simulink model "MotorGenerator2_Component_harness_model"  (R2023a)
settings: Solver=daessc  StartTime=0.0  StopTime=200  RelTol=1e-3  AbsTol=1e-3
PreLoadFcn:
  | MotorGenerator2_Component_harness_setup
undefined symbols (not defined in the file or in its folder): batteryHighVoltage, initial, Minus, motorGenerator2, Plus
libraries: fl_lib x18, nesl_utility x14, sdl_lib x1
settings Model: Creator=isaacito  LastModifiedBy=isaacito
settings SolverCC: AutoScaleAbsTol=off  AlgebraicLoopSolver=TrustRegion
settings DataIOCC: DSMLogging=off
settings OptimizationCC: ReuseModelBlockBuffer=off
settings DebuggingCC: UnconnectedInputMsg=warning  UnconnectedOutputMsg=warning  UnconnectedLineMsg=warning  SymbolicDimsDataTypeCodeGenerationDiagnostic=none
settings ModelReferenceCC: EnableRefExpFcnMdlSchedulingChecks=on
settings SFSimCC: CustomCodeUndefinedFunction=UseInterfaceOnly
settings RTWCC: DLArmComputeVersion=19.05
settings SimscapeCC: SimscapeLogType=all  SimscapeLogSimulationStatistics=on  SimscapeLogLimitData=off  SimscapeLogDataHistory=10000

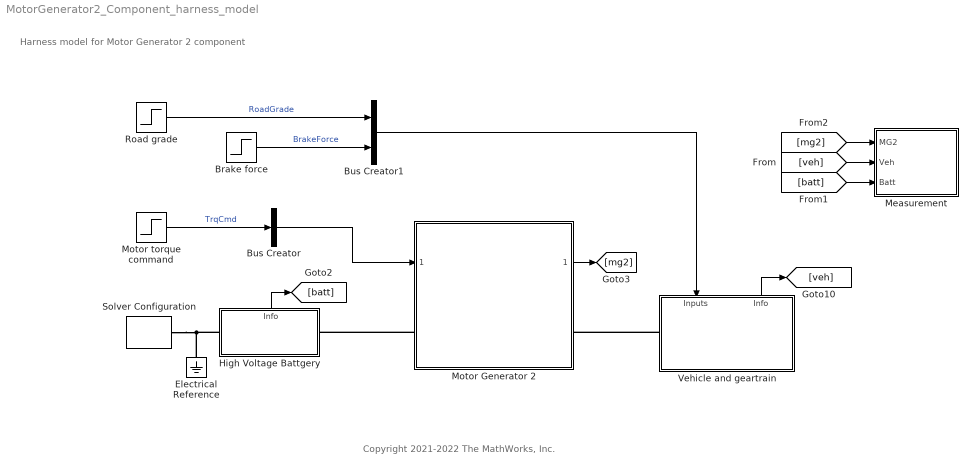
== system MotorGenerator2_Component_harness_model ==
  note: Copyright 2021-2022 The MathWorks, Inc.
  note: Harness model for Motor Generator 2 component
  Brake force : Step  After=0  SampleTime=0
      settings: AttributesFormatString=|
      | Before: %<Before>
      | Time: %<Time>
      | After: %<After>
  Bus Creator : BusCreator  Inputs=1
  Bus Creator1 : BusCreator  Inputs=2
  Electrical Reference : fl_lib/Electrical/Electrical Elements/Electrical Reference
  High Voltage Battgery : Subsystem
      settings: PortSchema="{\"entries\":[{\"content\":{\"sides\":[{\"content\":{\"connectorIds\":[\"LConn1\"]},\"type\":\"ConnectorPlacement.EquallySpacedRectSide\",\"uuid\":\"8acd7e9a-bb08-4de6-aa14-0989ebba81b9\"},{\"content\":{\"connectorIds\":[\"RConn1\"],\"side\":\"RIGHT\"},\"type\":\"ConnectorPlacement.EquallySpacedRectSide\",\"uuid\":\"f80e1afc-966f-4d6b-84f9-f0b60dd6f20c\"},{\"content\":{\"connectorIds\":[\"Out1\"],\"side\":\"TOP\"},\"type\":\"ConnectorPlacement.EquallySpacedRectSide\",\"uuid\":\"52ccb2b1-bd5e-4dcb-b9b6-0ef03b912c33\"}]},\"type\":\"ConnectorPlacement.EquallySpacedConnector\",\"uuid\":\"b55f48a4-f283-4a77-8513-99b31abb285a\"}],\"packageUris\":[\"http://schema.mathworks.com/mf0/Connector/R2020b\"],\"version\":\"1.0\"}"
  Measurement : Subsystem
  Motor Generator 2 : Subsystem  ReferencedSubsystem=MotorDriveUnit_refsub_Basic  torque_max=motorGenerator2.trqMax_Nm  Value=motorGenerator2.powerMax_kW  Tc=motorGenerator2.responseTime_s  eff=motorGenerator2.efficiency_pct  w_eff=motorGenerator2.spd_eff_rpm  T_eff=motorGenerator2.trq_eff_Nm  thermal_mass=motorGenerator2.thermalMass_J_perK  temperature=initial.MG2_Temperature_K  k=motorGenerator2.dampSpringStiffness_Nm_per_rad  mu_visc=motorGenerator2.dampSpringFriction_Nm_per_rpm  w_tol=smoothing.MG2_dampSpringVelTol_rpm  T=initial.MG2_AirTemp_K
      settings: PortSchema="{\"entries\":[{\"content\":{\"sides\":[{\"content\":{\"connectorIds\":[\"In1\",\"LConn1\"]},\"type\":\"ConnectorPlacement.EquallySpacedRectSide\",\"uuid\":\"02d16a10-ccfb-4288-a5a1-1144159c5ca2\"},{\"content\":{\"connectorIds\":[\"Out1\",\"LConn2\"],\"side\":\"RIGHT\"},\"type\":\"ConnectorPlacement.EquallySpacedRectSide\",\"uuid\":\"b2601986-efe5-4f5e-bd54-3f5cb03e9252\"},{\"content\":{\"connectorIds\":[],\"side\":\"TOP\"},\"type\":\"ConnectorPlacement.EquallySpacedRectSide\",\"uuid\":\"248805f0-4416-4f49-8b0b-c2d3fe77e89e\"}]},\"type\":\"ConnectorPlacement.EquallySpacedConnector\",\"uuid\":\"35449164-35fe-478e-9b2e-66e853caa6da\"}],\"packageUris\":[\"http://schema.mathworks.com/mf0/Connector/R2020b\"],\"version\":\"1.0\"}"
  Motor torque command : Step  Time=50  Before=50  After=100  SampleTime=0
      settings: AttributesFormatString=|
      | Before: %<Before>
      | Time: %<Time>
      | After: %<After>
  Road grade : Step  Time=100  After=7  SampleTime=0
      settings: AttributesFormatString=|
      | Before: %<Before>
      | Time: %<Time>
      | After: %<After>
  Solver Configuration : nesl_utility/Solver Configuration  PhysicalDomain=network_engine_domain  SubClassName=solver  LeftPortType=input  RightPortType=generic  Tones=[]  Harmonics=[]  SimulateNoise=off  Profile=off  UseLocalSampling=off  EnableSwitchedLinearOptims=on  FrequencyDomain=off  UseCCode=off  RelTol=0.001  AbsTol=1e-06  MinStep=1e-09  ToWorkspace=off  RevertToSquareIcSolve=off  NumHomotopyIterations=100  PhasorMode=off  PhasorModeNumHarmonics=1  ConsistencySolver=NEWTON_FTOL  IndexReductionMethod=DerivativeReplacement  DoDC=off  ResidualTolerance=1e-09  ConsistencyTolSource=GLOBAL  ConsistencyAbsTol=0.001  ConsistencyRelTol=0.001  ConsistencyTolFactor=0.001  UseLocalSolver=off  LocalSolverChoice=NE_BACKWARD_EULER_ADVANCER  ResolveIndetEquations=on  FunctionEvalNumThread=1  LocalSolverSampleTime=0.001  DoFixedCost=off  MaxNonlinIter=3  MaxModeIter=2  ComputeImpulses=off  ImpulseIterations=2  LinearAlgebra=auto  LinearAlgebraNumThread=0  EquationFormulation=NE_TIME_EF  DelaysMemoryBudget=1024  AutomaticFiltering=on  FilteringTimeConstant=0.001  PartitionStorageMethod=AS_NEEDED  PartitionMemoryBudget=1024  PartitionMethod=ROBUST
      settings: AttributesFormatString=Local solver %<UseLocalSolver>
  Vehicle and geartrain : Subsystem
      settings: PortSchema="{\"entries\":[{\"content\":{\"sides\":[{\"content\":{\"connectorIds\":[\"LConn1\"]},\"type\":\"ConnectorPlacement.EquallySpacedRectSide\",\"uuid\":\"26173f4b-7c8a-4f16-9397-bd2703a262c3\"},{\"content\":{\"connectorIds\":[],\"side\":\"RIGHT\"},\"type\":\"ConnectorPlacement.EquallySpacedRectSide\",\"uuid\":\"c1cca5f5-e160-4db7-9272-a3c788f9ef94\"},{\"content\":{\"connectorIds\":[\"In1\",\"Out1\"],\"side\":\"TOP\"},\"type\":\"ConnectorPlacement.EquallySpacedRectSide\",\"uuid\":\"12b52f59-061a-44b9-b00e-a084783c45fb\"}]},\"type\":\"ConnectorPlacement.EquallySpacedConnector\",\"uuid\":\"a6613901-d795-4b91-ba16-2f1b373021b5\"}],\"packageUris\":[\"http://schema.mathworks.com/mf0/Connector/R2020b\"],\"version\":\"1.0\"}"
  wires:
  High Voltage Battgery/1(Info) -> [batt]
  Motor Generator 2/1 -> [mg2]
  Vehicle and geartrain/1(Info) -> [veh]
  [veh] -> Measurement/2(Veh)
  [mg2] -> Measurement/1(MG2)
  [batt] -> Measurement/3(Batt)
  Motor torque command/1 -> Bus Creator/1  "TrqCmd"
  Bus Creator/1 -> Motor Generator 2/1
  Road grade/1 -> Bus Creator1/1  "RoadGrade"
  Brake force/1 -> Bus Creator1/2  "BrakeForce"
  Bus Creator1/1 -> Vehicle and geartrain/1(Inputs)
  connections:
  High Voltage Battgery/LConn1 -- Solver Configuration/RConn1 -- Electrical Reference/LConn1
  Motor Generator 2/LConn1 -- High Voltage Battgery/RConn1
  Vehicle and geartrain/LConn1 -- Motor Generator 2/LConn2

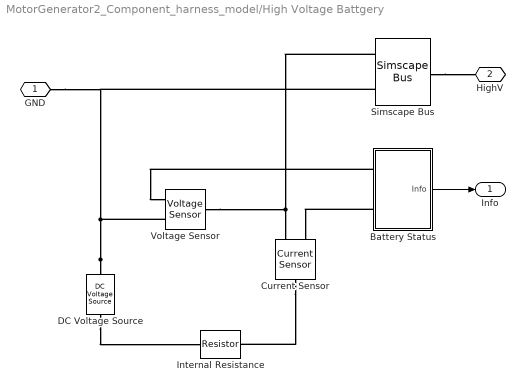
== system MotorGenerator2_Component_harness_model/High Voltage Battgery ==
  Battery Status : Subsystem
  Current Sensor : fl_lib/Electrical/Electrical Sensors/Current Sensor
  DC Voltage Source : fl_lib/Electrical/Electrical Sources/DC Voltage Source  v0=batteryHighVoltage.voltage_V V
      settings: AttributesFormatString=%<v0> [%<v0_unit>]
  Internal Resistance : fl_lib/Electrical/Electrical Elements/Resistor  R=batteryHighVoltage.internal_R_Ohm Ohm  i_specify=off  i_priority=High  i=0 A  i_nominal_specify=off  i_nominal_unit=A  i_nominal_value=1  v_specify=off  v_priority=High  v=0 V  v_nominal_specify=off  v_nominal_unit=V  v_nominal_value=1
      settings: AttributesFormatString=%<R> [%<R_unit>]
  Simscape Bus : SimscapeBus  HierarchyStrings=Plus;Minus  ConnectionType=Bus: Bus_HighVoltage
      settings: AttributesFormatString=%<ConnectionType>
  Voltage Sensor : fl_lib/Electrical/Electrical Sensors/Voltage Sensor
  GND : PMIOPort  Side=Left
  HighV : PMIOPort  Port=2  Side=Right
  Info : Outport
  wires:
  Battery Status/1(Info) -> Info/1
  connections:
  DC Voltage Source/RConn1 -- Simscape Bus/LConn2 -- GND/RConn1 -- Voltage Sensor/RConn2
  Simscape Bus/LConn1 -- Voltage Sensor/LConn1 -- Current Sensor/RConn2
  Battery Status/LConn2 -- Current Sensor/RConn1
  Simscape Bus/RConn1 -- HighV/RConn1
  Current Sensor/LConn1 -- Internal Resistance/RConn1
  DC Voltage Source/LConn1 -- Internal Resistance/LConn1
  Battery Status/LConn1 -- Voltage Sensor/RConn1

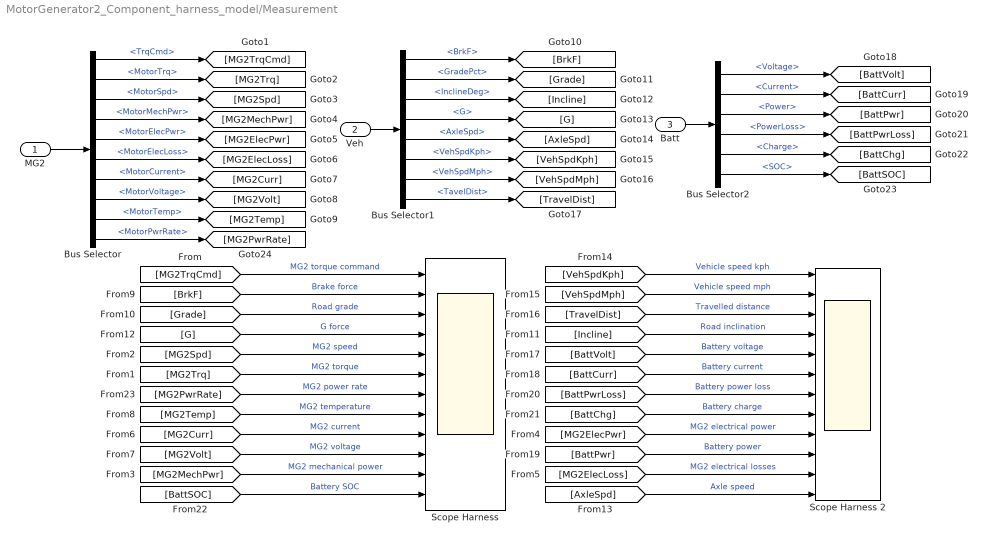
== system MotorGenerator2_Component_harness_model/Measurement ==
  MG2 : Inport
  Veh : Inport  Port=2
  Batt : Inport  Port=3
  Bus Selector : BusSelector  OutputSignals=TrqCmd,MotorTrq,MotorSpd,MotorMechPwr,MotorElecPwr,MotorElecLoss,MotorCurrent,MotorVoltage,MotorTemp,MotorPwrRate
  Bus Selector1 : BusSelector  OutputSignals=BrkF,GradePct,InclineDeg,G,AxleSpd,VehSpdKph,VehSpdMph,TavelDist
  Bus Selector2 : BusSelector  OutputSignals=Voltage,Current,Power,PowerLoss,Charge,SOC
  Scope Harness : Scope  NumInputPorts=12
  Scope Harness 2 : Scope  NumInputPorts=12
  wires:
  Veh/1 -> Bus Selector1/1
  MG2/1 -> Bus Selector/1
  Bus Selector/1 -> [MG2TrqCmd]  "<TrqCmd>"
  Bus Selector/2 -> [MG2Trq]  "<MotorTrq>"
  Bus Selector/3 -> [MG2Spd]  "<MotorSpd>"
  Bus Selector/4 -> [MG2MechPwr]  "<MotorMechPwr>"
  Bus Selector/5 -> [MG2ElecPwr]  "<MotorElecPwr>"
  Bus Selector/6 -> [MG2ElecLoss]  "<MotorElecLoss>"
  Bus Selector/7 -> [MG2Curr]  "<MotorCurrent>"
  Bus Selector/8 -> [MG2Volt]  "<MotorVoltage>"
  Bus Selector/9 -> [MG2Temp]  "<MotorTemp>"
  Batt/1 -> Bus Selector2/1
  Bus Selector1/1 -> [BrkF]  "<BrkF>"
  Bus Selector1/2 -> [Grade]  "<GradePct>"
  Bus Selector1/3 -> [Incline]  "<InclineDeg>"
  Bus Selector1/4 -> [G]  "<G>"
  Bus Selector1/5 -> [AxleSpd]  "<AxleSpd>"
  Bus Selector1/6 -> [VehSpdKph]  "<VehSpdKph>"
  Bus Selector1/7 -> [VehSpdMph]  "<VehSpdMph>"
  Bus Selector1/8 -> [TravelDist]  "<TavelDist>"
  Bus Selector2/1 -> [BattVolt]  "<Voltage>"
  Bus Selector2/2 -> [BattCurr]  "<Current>"
  Bus Selector2/3 -> [BattPwr]  "<Power>"
  Bus Selector2/4 -> [BattPwrLoss]  "<PowerLoss>"
  Bus Selector2/5 -> [BattChg]  "<Charge>"
  Bus Selector2/6 -> [BattSOC]  "<SOC>"
  [MG2TrqCmd] -> Scope Harness/1  "MG2 torque command"
  [BrkF] -> Scope Harness/2  "Brake force"
  [Grade] -> Scope Harness/3  "Road grade"
  [G] -> Scope Harness/4  "G force"
  [MG2Spd] -> Scope Harness/5  "MG2 speed"
  [MG2Trq] -> Scope Harness/6  "MG2 torque"
  [MG2Temp] -> Scope Harness/8  "MG2 temperature"
  [MG2Curr] -> Scope Harness/9  "MG2 current"
  [MG2Volt] -> Scope Harness/10  "MG2 voltage"
  [BattSOC] -> Scope Harness/12  "Battery SOC"
  [VehSpdKph] -> Scope Harness 2/1  "Vehicle speed kph"
  [VehSpdMph] -> Scope Harness 2/2  "Vehicle speed mph"
  [TravelDist] -> Scope Harness 2/3  "Travelled distance"
  [Incline] -> Scope Harness 2/4  "Road inclination"
  [BattVolt] -> Scope Harness 2/5  "Battery voltage"
  [BattCurr] -> Scope Harness 2/6  "Battery current"
  [BattPwrLoss] -> Scope Harness 2/7  "Battery power loss"
  [BattChg] -> Scope Harness 2/8  "Battery charge"
  [MG2ElecPwr] -> Scope Harness 2/9  "MG2 electrical power"
  Bus Selector/10 -> [MG2PwrRate]  "<MotorPwrRate>"
  [MG2PwrRate] -> Scope Harness/7  "MG2 power rate"
  [MG2MechPwr] -> Scope Harness/11  "MG2 mechanical power"
  [BattPwr] -> Scope Harness 2/10  "Battery power"
  [MG2ElecLoss] -> Scope Harness 2/11  "MG2 electrical losses"
  [AxleSpd] -> Scope Harness 2/12  "Axle speed"

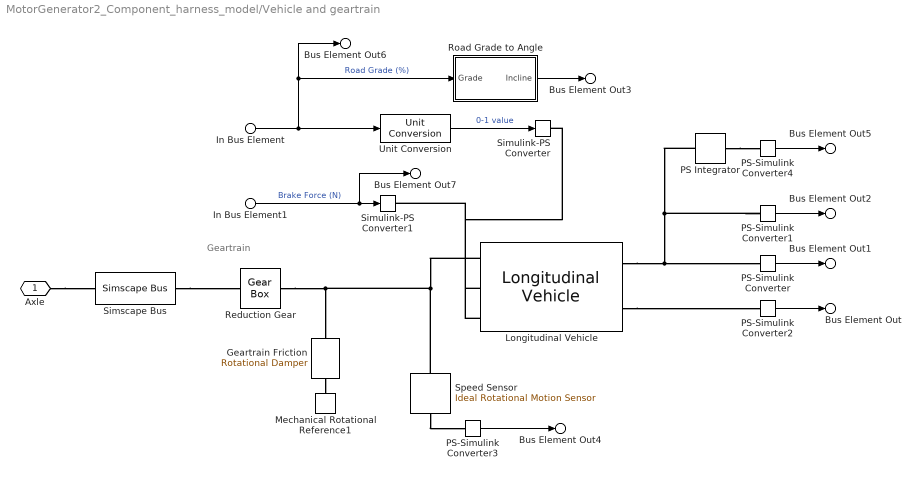
== system MotorGenerator2_Component_harness_model/Vehicle and geartrain ==
  note: Geartrain
  In Bus Element : Inport  PortName=Inputs  Element=RoadGrade
      settings: AttributesFormatString=%<Unit>
  In Bus Element1 : Inport  PortName=Inputs  Element=BrakeForce
      settings: AttributesFormatString=%<Unit>
  Geartrain Friction : fl_lib/Mechanical/Rotational Elements/Rotational Damper  D=0.01 m*N/rpm  w_specify=off  w_priority=None  w=0 rad/s  w_nominal_specify=off  w_nominal_unit=rad/s  w_nominal_value=1  t_specify=off  t_priority=None  t=0 N*m  t_nominal_specify=off  t_nominal_unit=N*m  t_nominal_value=1
      settings: AttributesFormatString=%<D> %<D_unit>
  Longitudinal Vehicle : sdl_lib/Tires & Vehicles/Longitudinal Vehicle  vehParamType=sdl.enum.VehicleParameterizationType.RoadLoad  M_vehicle=1200 kg  R_tireroll=0.3 m  C_tireroll=0.0136  C_airdrag=0.31  A_front=2.3 m^2  A_rl=120 N  B_rl=1.8 N/(m/s)  C_rl=0.389 N/(m/s)^2  g=9.81 m/s^2  V_1=0.3 m/s  w_1=0.01 rad/s  ShowBrakeIn=simscape.enum.onoff.on  ShowSlopeIn=simscape.enum.onoff.on  SlopeInputType=sdl.enum.VehicleLongitudinalRoadSlopeInputType.Grade  ShowWindIn=simscape.enum.onoff.off  ShowGOut=simscape.enum.onoff.on  air_density=1.184 kg/m^3  V_x_specify=on  V_x_priority=High  V_x=initial.vehicle_speed_kph km/hr  V_x_nominal_specify=off  V_x_nominal_unit=m/s  V_x_nominal_value=1  trq_specify=off  trq_priority=None  trq=0 N*m  trq_nominal_specify=off  trq_nominal_unit=N*m  trq_nominal_value=1  w_specify=off  w_priority=None  w=0 rad/s  w_nominal_specify=off  w_nominal_unit=rad/s  w_nominal_value=1
      settings: InternalSimscapePortConfiguration="{\"Bottom\":[],\"Left\":[{\"id\":\"Axle\",\"label\":\"Axle\",\"type\":\"foundation.mechanical.rotational.rotational\"}],\"Right\":[{\"id\":\"v_out\",\"label\":\"VehSpd\",\"type\":\"output\"},{\"id\":\"G_out\",\"label\":\"G\",\"type\":\"output\"}],\"Top\":[{\"id\":\"brkF\",\"label\":\"Brake\",\"type\":\"input\"},{\"id\":\"grade_norm\",\"label\":\"NG\",\"type\":\"input\"}]}"
      settings: AttributesFormatString=|
      | %<V_x> [%<V_x_unit>]
      | Priority: %<V_x_priority>
  Mechanical Rotational Reference1 : fl_lib/Mechanical/Rotational Elements/Mechanical Rotational Reference
  PS Integrator : fl_lib/Physical Signals/Linear Operators/PS Integrator  reset_method=foundation.enum.IntegratorResetSpec.None  initial_condition_spec=foundation.enum.IntegratorICSpec.Internal  saturation_spec=foundation.enum.IntegratorSaturationSpec.None  saturation_source_spec=foundation.enum.IntegratorSaturationSourceSpec.Internal  x0=0 km  xu=inf s  xl=-inf s
      settings: AttributesFormatString=Initial: %<x0> %<x0_unit>
  PS-Simulink Converter : nesl_utility/PS-Simulink Converter  PhysicalDomain=network_engine_domain  SubClassName=ps_output  LeftPortType=input  RightPortType=output  PseudoPeriodic=off  Frequencies=[]  VectorFormat=1-D array  Unit=km/hr  AffineConversion=off
  PS-Simulink Converter1 : nesl_utility/PS-Simulink Converter  PhysicalDomain=network_engine_domain  SubClassName=ps_output  LeftPortType=input  RightPortType=output  PseudoPeriodic=off  Frequencies=[]  VectorFormat=1-D array  Unit=mph  AffineConversion=off
  PS-Simulink Converter2 : nesl_utility/PS-Simulink Converter  PhysicalDomain=network_engine_domain  SubClassName=ps_output  LeftPortType=input  RightPortType=output  PseudoPeriodic=off  Frequencies=[]  VectorFormat=1-D array  Unit=1  AffineConversion=off
  PS-Simulink Converter3 : nesl_utility/PS-Simulink Converter  PhysicalDomain=network_engine_domain  SubClassName=ps_output  LeftPortType=input  RightPortType=output  PseudoPeriodic=off  Frequencies=[]  VectorFormat=1-D array  Unit=rpm  AffineConversion=off
  PS-Simulink Converter4 : nesl_utility/PS-Simulink Converter  PhysicalDomain=network_engine_domain  SubClassName=ps_output  LeftPortType=input  RightPortType=output  PseudoPeriodic=off  Frequencies=[]  VectorFormat=1-D array  Unit=km  AffineConversion=off
  Reduction Gear : fl_lib/Mechanical/Mechanisms/Gear Box  ratio=9  t_in_specify=off  t_in_priority=None  t_in=0 N*m  t_in_nominal_specify=off  t_in_nominal_unit=N*m  t_in_nominal_value=1  t_out_specify=off  t_out_priority=None  t_out=0 N*m  t_out_nominal_specify=off  t_out_nominal_unit=N*m  t_out_nominal_value=1
      settings: AttributesFormatString=%<ratio>
  Road Grade to Angle : Subsystem
  Simscape Bus : SimscapeBus  HierarchyStrings=AngSpd  ConnectionType=Bus: Bus_Rotational
      settings: AttributesFormatString=%<ConnectionType>
  Simulink-PS Converter : nesl_utility/Simulink-PS Converter  PhysicalDomain=network_engine_domain  SubClassName=ps_input  LeftPortType=input  RightPortType=output  PseudoPeriodic=off  Frequencies=[]  NoiseDistribution=none  NoiseParameters=[]  Unit=1  AffineConversion=off  FilteringAndDerivatives=filter  SimscapeFilterOrder=1  InputFilterTimeConstant=0.001  UdotUserProvided=0
  Simulink-PS Converter1 : nesl_utility/Simulink-PS Converter  PhysicalDomain=network_engine_domain  SubClassName=ps_input  LeftPortType=input  RightPortType=output  PseudoPeriodic=off  Frequencies=[]  NoiseDistribution=none  NoiseParameters=[]  Unit=N  AffineConversion=off  FilteringAndDerivatives=filter  SimscapeFilterOrder=1  InputFilterTimeConstant=0.001  UdotUserProvided=0
  Speed Sensor : fl_lib/Mechanical/Mechanical Sensors/Ideal Rotational Motion Sensor  reference=foundation.enum.MeasurementReference.absolute  acceleration_port=false  velocity_port=true  position_port=false  wrap_angle=simscape.enum.onoff.off  offset=0 rad
      settings: InternalSimscapePortConfiguration="{\"Bottom\":[],\"Left\":[{\"id\":\"R\",\"label\":\"R\",\"type\":\"foundation.mechanical.rotational.rotational\"}],\"Right\":[{\"id\":\"W\",\"label\":\"W\",\"type\":\"output\"}],\"Top\":[]}"
  Unit Conversion : UnitConversion  OutputType=Inherit: Inherit via back propagation
  Axle : PMIOPort  Side=Left
  Bus Element Out : Outport  PortName=Info  Element=G
      settings: AttributesFormatString=%<Unit>
  Bus Element Out1 : Outport  PortName=Info  Element=VehSpdKph
      settings: AttributesFormatString=%<Unit>
  Bus Element Out2 : Outport  PortName=Info  Element=VehSpdMph
      settings: AttributesFormatString=%<Unit>
  Bus Element Out3 : Outport  PortName=Info  Element=InclineDeg
      settings: AttributesFormatString=%<Unit>
  Bus Element Out4 : Outport  PortName=Info  Element=AxleSpd
      settings: AttributesFormatString=%<Unit>
  Bus Element Out5 : Outport  PortName=Info  Element=TavelDist
      settings: AttributesFormatString=%<Unit>
  Bus Element Out6 : Outport  PortName=Info  Element=GradePct
      settings: AttributesFormatString=%<Unit>
  Bus Element Out7 : Outport  PortName=Info  Element=BrkF
      settings: AttributesFormatString=%<Unit>
  wires:
  PS-Simulink Converter1/1 -> Bus Element Out2/1
  Unit Conversion/1 -> Simulink-PS Converter/1  "0-1 value"
  In Bus Element1/1 -> Bus Element Out7/1, Simulink-PS Converter1/1  "Brake Force (N)"
  PS-Simulink Converter3/1 -> Bus Element Out4/1
  PS-Simulink Converter/1 -> Bus Element Out1/1
  In Bus Element/1 -> Bus Element Out6/1, Road Grade to Angle/1(Grade), Unit Conversion/1  "Road Grade (%)"
  PS-Simulink Converter2/1 -> Bus Element Out/1
  Road Grade to Angle/1(Incline) -> Bus Element Out3/1
  PS-Simulink Converter4/1 -> Bus Element Out5/1
  connections:
  Longitudinal Vehicle/RConn1 -- PS Integrator/LConn1 -- PS-Simulink Converter1/LConn1 -- PS-Simulink Converter/LConn1
  Longitudinal Vehicle/LConn2 -- Simulink-PS Converter1/RConn1
  Longitudinal Vehicle/LConn3 -- Simulink-PS Converter/RConn1
  Speed Sensor/RConn1 -- PS-Simulink Converter3/LConn1
  Longitudinal Vehicle/RConn2 -- PS-Simulink Converter2/LConn1
  Reduction Gear/RConn1 -- Speed Sensor/LConn1 -- Longitudinal Vehicle/LConn1 -- Geartrain Friction/LConn1
  Simscape Bus/LConn1 -- Reduction Gear/LConn1
  Geartrain Friction/RConn1 -- Mechanical Rotational Reference1/LConn1
  Axle/RConn1 -- Simscape Bus/RConn1
  PS Integrator/RConn1 -- PS-Simulink Converter4/LConn1

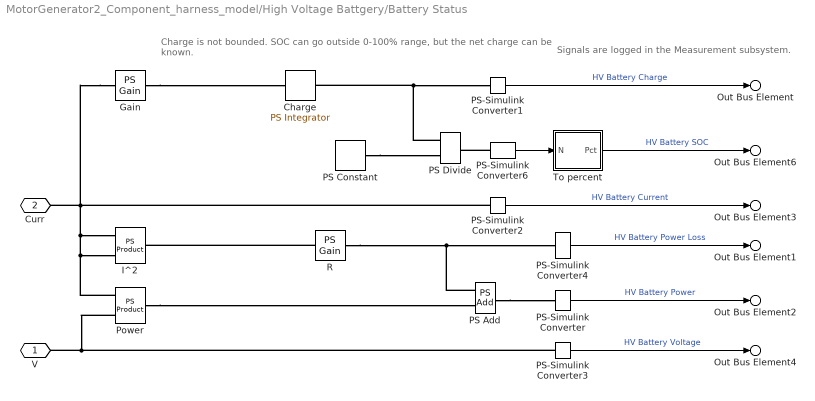
== system MotorGenerator2_Component_harness_model/High Voltage Battgery/Battery Status ==
  note: Signals are logged in the Measurement subsystem.
  note: Charge is not bounded. SOC can go outside 0-100% range,
      | but the net charge can be known.
  Charge : fl_lib/Physical Signals/Linear Operators/PS Integrator  reset_method=foundation.enum.IntegratorResetSpec.None  initial_condition_spec=foundation.enum.IntegratorICSpec.Internal  saturation_spec=foundation.enum.IntegratorSaturationSpec.None  saturation_source_spec=foundation.enum.IntegratorSaturationSourceSpec.Internal  x0=initial.hvBattery_Charge_Ahr A*hr  xu=inf s  xl=-inf s
      settings: AttributesFormatString=%<x0> [%<x0_unit>]
  Gain : fl_lib/Physical Signals/Functions/PS Gain  gain=-1
      settings: AttributesFormatString=%<gain>
  I^2 : fl_lib/Physical Signals/Functions/PS Product
  PS Add : fl_lib/Physical Signals/Functions/PS Add
  PS Constant : fl_lib/Physical Signals/Sources/PS Constant  constant=batteryHighVoltage.charge_Ahr A*hr
      settings: AttributesFormatString=%<constant> [%<constant_unit>]
  PS Divide : fl_lib/Physical Signals/Functions/PS Divide
  PS-Simulink Converter : nesl_utility/PS-Simulink Converter  PhysicalDomain=network_engine_domain  SubClassName=ps_output  LeftPortType=input  RightPortType=output  PseudoPeriodic=off  Frequencies=[]  VectorFormat=1-D array  Unit=kW  AffineConversion=off
  PS-Simulink Converter1 : nesl_utility/PS-Simulink Converter  PhysicalDomain=network_engine_domain  SubClassName=ps_output  LeftPortType=input  RightPortType=output  PseudoPeriodic=off  Frequencies=[]  VectorFormat=1-D array  Unit=A*hr  AffineConversion=off
  PS-Simulink Converter2 : nesl_utility/PS-Simulink Converter  PhysicalDomain=network_engine_domain  SubClassName=ps_output  LeftPortType=input  RightPortType=output  PseudoPeriodic=off  Frequencies=[]  VectorFormat=1-D array  Unit=A  AffineConversion=off
  PS-Simulink Converter3 : nesl_utility/PS-Simulink Converter  PhysicalDomain=network_engine_domain  SubClassName=ps_output  LeftPortType=input  RightPortType=output  PseudoPeriodic=off  Frequencies=[]  VectorFormat=1-D array  Unit=V  AffineConversion=off
  PS-Simulink Converter4 : nesl_utility/PS-Simulink Converter  PhysicalDomain=network_engine_domain  SubClassName=ps_output  LeftPortType=input  RightPortType=output  PseudoPeriodic=off  Frequencies=[]  VectorFormat=1-D array  Unit=W  AffineConversion=off
  PS-Simulink Converter6 : nesl_utility/PS-Simulink Converter  PhysicalDomain=network_engine_domain  SubClassName=ps_output  LeftPortType=input  RightPortType=output  PseudoPeriodic=off  Frequencies=[]  VectorFormat=1-D array  Unit=1  AffineConversion=off
  Power : fl_lib/Physical Signals/Functions/PS Product
  R : fl_lib/Physical Signals/Functions/PS Gain  gain=batteryHighVoltage.internal_R_Ohm Ohm
      settings: AttributesFormatString=%<gain> [%<gain_unit>]
  To percent : Subsystem
  V : PMIOPort  Side=Left
  Curr : PMIOPort  Port=2  Side=Left
  Out Bus Element : Outport  PortName=Info  Element=Charge
      settings: AttributesFormatString=%<Unit>
  Out Bus Element3 : Outport  PortName=Info  Element=Current
      settings: AttributesFormatString=%<Unit>
  Out Bus Element1 : Outport  PortName=Info  Element=PowerLoss
      settings: AttributesFormatString=%<Unit>
  Out Bus Element2 : Outport  PortName=Info  Element=Power
      settings: AttributesFormatString=%<Unit>
  Out Bus Element4 : Outport  PortName=Info  Element=Voltage
      settings: AttributesFormatString=%<Unit>
  Out Bus Element6 : Outport  PortName=Info  Element=SOC
      settings: AttributesFormatString=%<Unit>
  wires:
  PS-Simulink Converter6/1 -> To percent/1(N)
  To percent/1(Pct) -> Out Bus Element6/1  "HV Battery SOC"
  PS-Simulink Converter3/1 -> Out Bus Element4/1  "HV Battery Voltage"
  PS-Simulink Converter2/1 -> Out Bus Element3/1  "HV Battery Current"
  PS-Simulink Converter4/1 -> Out Bus Element1/1  "HV Battery Power Loss"
  PS-Simulink Converter1/1 -> Out Bus Element/1  "HV Battery Charge"
  PS-Simulink Converter/1 -> Out Bus Element2/1  "HV Battery Power"
  connections:
  PS-Simulink Converter6/LConn1 -- PS Divide/RConn1
  Power/RConn1 -- PS Add/LConn2
  PS Constant/RConn1 -- PS Divide/LConn2
  PS Add/RConn1 -- PS-Simulink Converter/LConn1
  R/LConn1 -- I^2/RConn1
  PS Divide/LConn1 -- PS-Simulink Converter1/LConn1 -- Charge/RConn1
  Gain/RConn1 -- Charge/LConn1
  PS Add/LConn1 -- PS-Simulink Converter4/LConn1 -- R/RConn1
  Power/LConn1 -- PS-Simulink Converter3/LConn1 -- V/RConn1
  Gain/LConn1 -- PS-Simulink Converter2/LConn1 -- Curr/RConn1 -- I^2/LConn1 -- Power/LConn2 -- I^2/LConn2

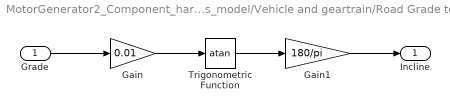
== system MotorGenerator2_Component_harness_model/Vehicle and geartrain/Road Grade to Angle ==
  Grade : Inport  Unit=%
      settings: AttributesFormatString=%<Unit>
  Gain : Gain  Gain=0.01
  Gain1 : Gain  Gain=180/pi
  Trigonometric Function : Trigonometry  Operator=atan
  Incline : Outport  Unit=deg
      settings: AttributesFormatString=%<Unit>
  wires:
  Gain/1 -> Trigonometric Function/1
  Grade/1 -> Gain/1
  Trigonometric Function/1 -> Gain1/1
  Gain1/1 -> Incline/1

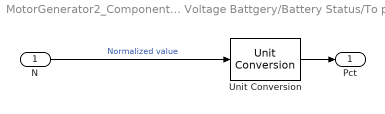
== system MotorGenerator2_Component_harness_model/High Voltage Battgery/Battery Status/To percent ==
  N : Inport
  Unit Conversion : UnitConversion
  Pct : Outport  Unit=%
      settings: AttributesFormatString=%<Unit>
  wires:
  N/1 -> Unit Conversion/1  "Normalized value"
  Unit Conversion/1 -> Pct/1
